simulink model "ecu_wifg"  (R2026a)
settings: Solver=FixedStepDiscrete  StopTime=10  FixedStep=0.001  SampleTimeConstraint=STIndependent
Description:
  | Water-in-fuel debounce. Source of truth for firmware/gen/ecu_wifg.
settings Model: Creator=jj1001000  LastModifiedBy=jj1001000
settings OptimizationCC: DefaultUnderspecifiedDataType=single
settings DebuggingCC: ParameterPrecisionLossMsg=none
settings HardwareCC: ProdLargestAtomicInteger=Long  ProdLargestAtomicFloat=Double  ProdHWDeviceType=ARM Compatible->ARM Cortex-M
settings RTWCC: SystemTargetFile=ert.tlc  GenCodeOnly=on  Description=Embedded Coder
settings ERTTargetCC: UtilityFuncGeneration=Shared location  IncludeMdlTerminateFcn=off  CodeInterfacePackaging=Reusable function  SupportNonFinite=off

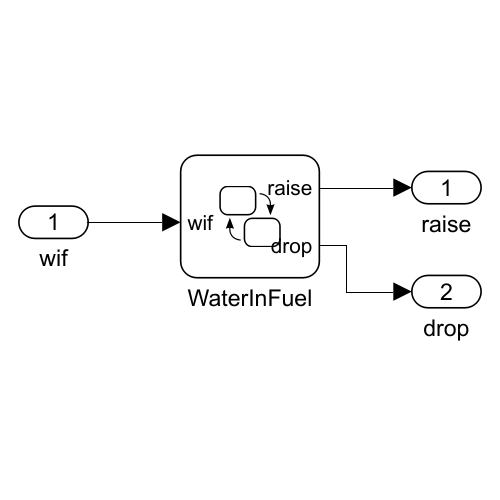
[thumbnail: Simulink's stored preview of the top-level diagram]
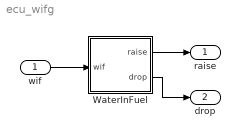
== system ecu_wifg ==
  wif : Inport  OutDataTypeStr=uint8
  WaterInFuel : Stateflow chart  TreatAsAtomicUnit=on
  raise : Outport  OutDataTypeStr=uint8
  drop : Outport  Port=2  OutDataTypeStr=uint8
  wires:
  wif/1 -> WaterInFuel/1(wif)
  WaterInFuel/1(raise) -> raise/1
  WaterInFuel/2(drop) -> drop/1

== stateflow chart ecu_wifg/WaterInFuel ==
  settings: updateMethod=DISCRETE  executeAtInitialization=1
  state DRYING
    entry: raise = uint8(0); drop = uint8(0);
    during: n = n + 1;
  state WETTING
    entry: raise = uint8(0); drop = uint8(0);
    during: n = n + 1;
  state DRY
    entry: raise = uint8(0); drop = uint8(1);
  state WET
    entry: raise = uint8(1); drop = uint8(0);
  (default) -> DRYING : {n = uint16(0); raise = uint8(0); drop = uint8(0);}
  DRYING -> WETTING [order 1] : [wif ~= 0]{n = uint16(1);}
  WETTING -> DRYING [order 1] : [wif == 0]{n = uint16(1);}
  DRYING -> DRY [order 2] : [n + 1 >= uint16(2000)]
  WET -> DRYING : [wif == 0]{n = uint16(1);}
  DRY -> WETTING : [wif ~= 0]{n = uint16(1);}
  WETTING -> WET [order 2] : [n + 1 >= uint16(2000)]
  data: wif input uint8; raise output uint8; drop output uint8; n local uint16
